simulink model "HouseHeating"  (R2026b)
settings: Solver=FixedStepAuto  StopTime=86400  FixedStep=1  AbsTol=1e-6
InitFcn:
  | sldemo_househeat_data
undefined symbols (not defined in the file): c_air, HeaterAirFlow, LRoof, LWall, LWindow, THeater, TinIC
libraries: fl_lib x22, nesl_utility x4
settings Model: ExtModeTrigMode=oneshot  Creator=The MathWorks, Inc.  LastModifiedBy=jolson
settings SolverCC: AutoScaleAbsTol=off
settings DataIOCC: ExternalInput=[]  InitialState=[]
settings OptimizationCC: BooleansAsBitfields=on  DataBitsets=on  DefaultParameterBehavior=Inlined  DifferentSizesBufferReuse=on  EfficientFloat2IntCast=on  EfficientTunableParamExpr=on  EnhancedBackFolding=on  GainParamInheritBuiltInType=on  InlineInvariantSignals=on  LifeSpan=1  NoFixptDivByZeroProtection=on  OptimizeBlockOrder=speed  PassReuseOutputArgsAs=Individual arguments  RemoveInternalMemoryZeroInit=on  RemoveRootLevelIOMemoryZeroInit=on  StateBitsets=on  UseDivisionForNetSlopeComputation=on  UseFloatMulNetSlope=on
settings DebuggingCC: ArithmeticOperatorsInVariantConditions=warning  BusObjectLabelMismatch=none  FcnCallInpInsideContextMsg=warning  IntegerOverflowMsg=none  IntegerSaturationMsg=none  MergeDetectMultiDrivingBlocksExec=none  MultiTaskCondExecSysMsg=none  MultiTaskDSMMsg=warning  ParameterTunabilityLossMsg=error  SFExecutionAtInitializationDiag=none  SFNoUnconditionalDefaultTransitionDiag=warning  SFUnexpectedBacktrackingDiag=warning  SaveWithParameterizedLinksMsg=none  SignalResolutionControl=TryResolveAllWithWarning  StateNameClashWarn=warning
settings HardwareCC: ProdEndianess=Unspecified  ProdEqTarget=off  ProdHWDeviceType=Generic->32-bit Embedded Processor  ProdIntDivRoundTo=Undefined  ProdLargestAtomicFloat=None  TargetEndianess=LittleEndian  TargetHWDeviceType=MATLAB Host  TargetIntDivRoundTo=Zero  TargetLongLongMode=on
settings ModelReferenceCC: PropagateSignalLabelsOutOfModel=off
settings SFSimCC: CustomCodeUndefinedFunction=UseInterfaceOnly  MATLABDynamicMemAlloc=off  SimUseLocalCustomCode=off
settings RTWCC: DataTypeReplacement=CDataTypesFixedWidth  Description=Embedded Coder  GenerateCodeMetricsReport=on  GenerateReport=on  GenerateTraceInfo=on  GenerateTraceReport=on  GenerateTraceReportEml=on  GenerateTraceReportSf=on  GenerateTraceReportSl=on  IncludeHyperlinkInReport=on  RTWUseLocalCustomCode=off  SystemTargetFile=ert.tlc  TemplateMakefile=ert_default_tmf
settings CodeAppCC: CustomSymbolStrFcn=$N$M$F  CustomSymbolStrGlobalVar=rt$N$M  CustomSymbolStrMacro=$N$M  CustomSymbolStrType=$N$M  ForceParamTrailComments=on  IgnoreCustomStorageClasses=off  InsertBlockDesc=on  OperatorAnnotations=on  SFDataObjDesc=on  SimulinkDataObjDesc=on
settings ERTTargetCC: CombineSignalStateStructs=on  GenerateSampleERTMain=on  MaxIdInt16=INT16_MAX  MaxIdInt32=INT32_MAX  MaxIdInt64=INT64_MAX  MaxIdInt8=INT8_MAX  MaxIdUint16=UINT16_MAX  MaxIdUint32=UINT32_MAX  MaxIdUint64=UINT64_MAX  MaxIdUint8=UINT8_MAX  MinIdInt16=INT16_MIN  MinIdInt32=INT32_MIN  MinIdInt64=INT64_MIN  MinIdInt8=INT8_MIN  SupportContinuousTime=on  SupportNonInlinedSFcns=on  SupportVariableSizeSignals=on
settings ConfigComp: CovExternalEMLEnable=off  CovSaveCumulativeToWorkspaceVar=on  CovSaveSingleToWorkspaceVar=on
settings SimscapeCC: SimscapeNominalValues="[{\"value\":\"1\",\"unit\":\"A\"},{\"value\":\"1\",\"unit\":\"bar\"},{\"value\":\"1\",\"unit\":\"cm^2\"},{\"value\":\"1\",\"unit\":\"cm^3/s\"},{\"value\":\"1\",\"unit\":\"kJ/kg\"},{\"value\":\"1\",\"unit\":\"kW\"},{\"value\":\"1\",\"unit\":\"l\"},{\"value\":\"1\",\"unit\":\"N\"},{\"value\":\"1\",\"unit\":\"N*m\"},{\"value\":\"1\",\"unit\":\"V\"},{\"value\":\"0.001\",\"unit\":\"Wb\"}]"  SimscapeUseEnergyAccounting=off

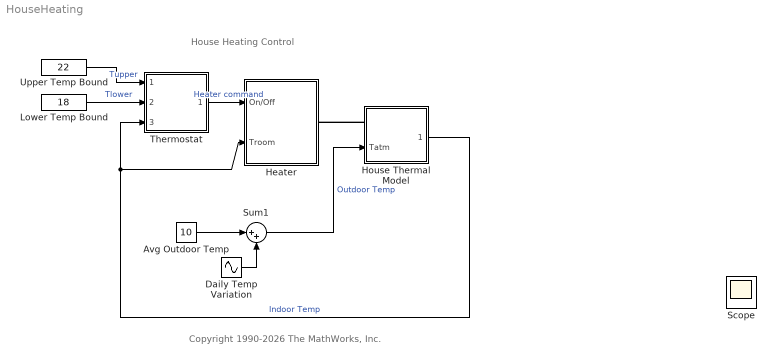
== system HouseHeating ==
  note: House Heating Control
  note: Copyright 1990-2026 The MathWorks, Inc.
  Avg Outdoor Temp : Constant  Value=10
  Daily Temp Variation : Sin  Amplitude=8  Frequency=(2*pi)/(24*3600)  Phase=-pi/2  SampleTime=0
  Heater : Subsystem
  House Thermal Model : Subsystem  Tag=PublishSubsystem
      settings: PortSchema="{\"entries\":[{\"content\":{\"sides\":[{\"content\":{\"connectorIds\":[\"LConn1\",\"In1\"]},\"type\":\"ConnectorPlacement.EquallySpacedRectSide\",\"uuid\":\"eb8069c2-07b2-4f5c-b9f9-5056c4795f4a\"},{\"content\":{\"connectorIds\":[\"Out1\"],\"side\":\"RIGHT\"},\"type\":\"ConnectorPlacement.EquallySpacedRectSide\",\"uuid\":\"80b7e6ec-7098-4e9e-918e-5666993f77ee\"},{\"content\":{\"side\":\"TOP\"},\"type\":\"ConnectorPlacement.EquallySpacedRectSide\",\"uuid\":\"1688e31c-8726-4a54-817f-3a69db3dd392\"}]},\"type\":\"ConnectorPlacement.EquallySpacedConnector\",\"uuid\":\"cc8e1f79-9fa5-412b-9d41-2aa535beff48\"}],\"packageUris\":[\"http://schema.mathworks.com/mf0/Connector/R2020b\"],\"version\":\"1.0\"}"
      mask Display:
      | plot([99.4454661849886;170.309218810871;170.309218810871;99.4454661849886;99.4454661849886], [212.827470386401;212.827470386401;127.790967235342;127.790967235342;212.827470386401])
      | plot([99.4454661849886;170.309218810871], [184.481969336048;184.481969336048])
      | plot([133.460067445412;133.460067445412], [184.481969336048;127.790967235342])
      | plot([241.172971436754;312.036724062636;312.036724062636;241.172971436754;241.172971436754], [212.827470386401;212.827470386401;127.790967235342;127.790967235342;212.827470386401])
      | plot([241.172971436754;312.036724062636], [184.481969336048;184.481969336048])
      | plot([275.187572697178;275.187572697178], [184.481969336048;127.790967235342])
      | plot([113.618216710165;42.7544640842825;368.727726163343;428.253278369084], [453.764229314402;255.34572196193;255.34572196193;453.764229314402])
      | plot([428.253278369084;499.117030994967], [453.764229314402;382.900476688519])
      | plot([113.618216710165;428.253278369084], [453.764229314402;453.764229314402])
      | plot([498.86507098563;499.368991004303], [382.900476688519;382.900476688519])
      | plot([482.109730364755;496.282480889931], [382.900476688519;382.900476688519])
      | plot([482.109730364755;374.396826373413], [382.900476688519;275.187572697178])
      | plot([482.109730364755;425.418728264049], [382.900476688519;439.591478789225])
      | plot([56.927214609459;56.927214609459;354.554975638166], [255.34572196193;56.927214609459;56.927214609459])
      | plot([354.554975638166;354.554975638166], [56.927214609459;255.34572196193])
      | plot([354.554975638166;482.109730364755;482.109730364755], [56.927214609459;184.481969336048;382.900476688519])
      | plot([397.073227213696;397.073227213696;439.591478789225;439.591478789225;397.073227213696], [170.309218810871;255.34572196193;297.86397353746;209.992920281366;170.309218810871])
      | plot([397.073227213696;439.591478789225], [227.000220911577;269.518472487107])
      | plot([419.749628053978;419.749628053978], [246.842071646824;192.985619651154])
      | %patch([0;553.20969549939;553.20969549939;0;0;0.472425017505884;0.47242501750577;552.737270481884;552.737270481885;0.472425017505884;0], [496.518693398684;496.518693398684;0;0;496.518693398684;496.046268381178;0.472425017505884;0.472425017505884;496.046268381178;496.046268381178;496.518693398684], [1;1;1])
  Lower Temp Bound : Constant  Value=18
  Sum1 : Sum  Inputs=|++  InputSameDT=on  SaturateOnIntegerOverflow=on  OutDataTypeStr=Inherit: Same as first input
  Thermostat : Subsystem
  Upper Temp Bound : Constant  Value=22
  Scope : Scope
      settings: ActiveDisplayYMinimum=-0.49999999999999956  ActiveDisplayYMaximum=24.5
  wires:
  Thermostat/1(HeaterSwitch) -> Heater/1(On/Off)  "Heater command"
  Daily Temp Variation/1 -> Sum1/2
  Sum1/1 -> House Thermal Model/1(Tatm)  "Outdoor Temp"
  Avg Outdoor Temp/1 -> Sum1/1
  House Thermal Model/1(Troom) -> Thermostat/3(Thouse), Heater/2(Troom)  "Indoor Temp"
  Lower Temp Bound/1 -> Thermostat/2(Tlower)  "Tlower"
  Upper Temp Bound/1 -> Thermostat/1(Tupper)  "Tupper"
  connections:
  House Thermal Model/LConn1 -- Heater/RConn1

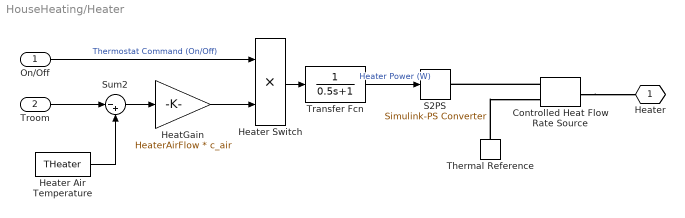
== system HouseHeating/Heater ==
  On/Off : Inport
  Troom : Inport  Port=2
  Controlled Heat Flow Rate Source : fl_lib/Thermal/Thermal Sources/Controlled Heat Flow Rate Source
  HeatGain : Gain  Gain=HeaterAirFlow * c_air
  Heater Air Temperature : Constant  Value=THeater
  Heater Switch : Product  RndMeth=Zero
  S2PS : nesl_utility/Simulink-PS Converter  PhysicalDomain=network_engine_domain  SubClassName=ps_input  LeftPortType=input  RightPortType=output  PseudoPeriodic=off  Frequencies=[]  NoiseDistribution=none  NoiseParameters=[]  Unit=1  AffineConversion=off  FilteringAndDerivatives=zero  SimscapeFilterOrder=1  InputFilterTimeConstant=.001  UdotUserProvided=0
  Sum2 : Sum  Inputs=|-+
  Thermal Reference : fl_lib/Thermal/Thermal Elements/Thermal Reference
  Transfer Fcn : TransferFcn  Denominator=[0.5 1]
  Heater : PMIOPort  Tag=PMCPort  Side=Right
  wires:
  Heater Air Temperature/1 -> Sum2/2
  Troom/1 -> Sum2/1
  Sum2/1 -> HeatGain/1
  On/Off/1 -> Heater Switch/1  "Thermostat Command (On/Off)"
  HeatGain/1 -> Heater Switch/2
  Heater Switch/1 -> Transfer Fcn/1
  Transfer Fcn/1 -> S2PS/1  "Heater Power (W)"
  connections:
  Controlled Heat Flow Rate Source/RConn1 -- S2PS/RConn1
  Thermal Reference/LConn1 -- Controlled Heat Flow Rate Source/RConn2
  Controlled Heat Flow Rate Source/LConn1 -- Heater/RConn1

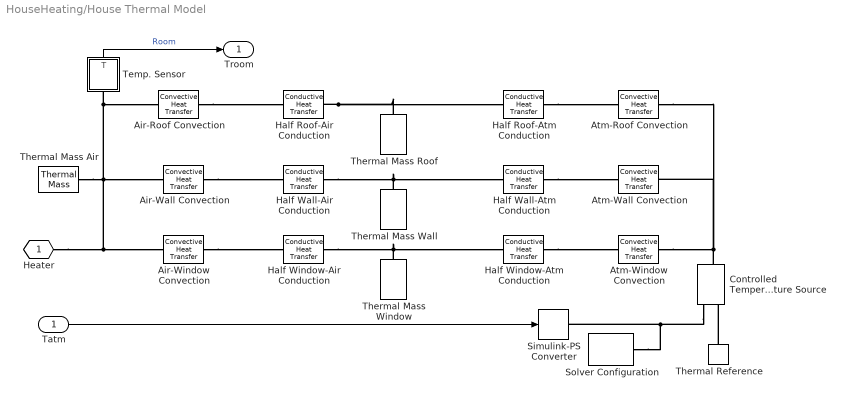
== system HouseHeating/House Thermal Model ==
  Tatm : Inport
  Air-Roof Convection : fl_lib/Thermal/Thermal Elements/Convective Heat Transfer  thermal_type=foundation.enum.constant_variable.constant  area=roofArea m^2  heat_tr_coeff=h_A_R W/m^2/K  min_heat_tr_coeff=1e-3 W/(K*m^2)  T_specify=off  T_priority=High  T=0 K  T_nominal_specify=off  T_nominal_value=1  T_nominal_unit=K  Q_specify=off  Q_priority=High  Q=0 J/s  Q_nominal_specify=off  Q_nominal_value=1  Q_nominal_unit=W
  Air-Wall Convection : fl_lib/Thermal/Thermal Elements/Convective Heat Transfer  thermal_type=foundation.enum.constant_variable.constant  area=wallArea m^2  heat_tr_coeff=h_A_W W/m^2/K  min_heat_tr_coeff=1e-3 W/(K*m^2)  T_specify=off  T_priority=High  T=0 K  T_nominal_specify=off  T_nominal_value=1  T_nominal_unit=K  Q_specify=off  Q_priority=High  Q=0 J/s  Q_nominal_specify=off  Q_nominal_value=1  Q_nominal_unit=W
  Air-Window Convection : fl_lib/Thermal/Thermal Elements/Convective Heat Transfer  thermal_type=foundation.enum.constant_variable.constant  area=windowArea m^2  heat_tr_coeff=h_A_Wnd W/m^2/K  min_heat_tr_coeff=1e-3 W/(K*m^2)  T_specify=off  T_priority=High  T=0 K  T_nominal_specify=off  T_nominal_value=1  T_nominal_unit=K  Q_specify=off  Q_priority=High  Q=0 J/s  Q_nominal_specify=off  Q_nominal_value=1  Q_nominal_unit=W
  Atm-Roof Convection : fl_lib/Thermal/Thermal Elements/Convective Heat Transfer  thermal_type=foundation.enum.constant_variable.constant  area=roofArea m^2  heat_tr_coeff=h_R_Atm W/m^2/K  min_heat_tr_coeff=1e-3 W/(K*m^2)  T_specify=off  T_priority=High  T=0 K  T_nominal_specify=off  T_nominal_value=1  T_nominal_unit=K  Q_specify=off  Q_priority=High  Q=0 J/s  Q_nominal_specify=off  Q_nominal_value=1  Q_nominal_unit=W
  Atm-Wall Convection : fl_lib/Thermal/Thermal Elements/Convective Heat Transfer  thermal_type=foundation.enum.constant_variable.constant  area=wallArea m^2  heat_tr_coeff=h_W_Atm W/m^2/K  min_heat_tr_coeff=1e-3 W/(K*m^2)  T_specify=off  T_priority=High  T=0 K  T_nominal_specify=off  T_nominal_value=1  T_nominal_unit=K  Q_specify=off  Q_priority=High  Q=0 J/s  Q_nominal_specify=off  Q_nominal_value=1  Q_nominal_unit=W
  Atm-Window Convection : fl_lib/Thermal/Thermal Elements/Convective Heat Transfer  thermal_type=foundation.enum.constant_variable.constant  area=windowArea m^2  heat_tr_coeff=h_Wnd_Atm W/m^2/K  min_heat_tr_coeff=1e-3 W/(K*m^2)  T_specify=off  T_priority=High  T=0 K  T_nominal_specify=off  T_nominal_value=1  T_nominal_unit=K  Q_specify=off  Q_priority=High  Q=0 J/s  Q_nominal_specify=off  Q_nominal_value=1  Q_nominal_unit=W
  Controlled Temperature Source : fl_lib/Thermal/Thermal Sources/Controlled Temperature Source
  Half Roof-Air Conduction : fl_lib/Thermal/Thermal Elements/Conductive Heat Transfer  thermal_type=foundation.enum.ConstantVariableTabulated.Constant  wall_geometry=foundation.enum.ConductionWallGeometry.Planar  area=roofArea m^2  thickness=LRoof/2 m  d_in=0.05 m  d_out=0.1 m  L=1 m  th_cond_min=10 W/(K*m)  th_cond=kRoof W/m/K  th_cond_TLU=[413, 401, 392, 383, 371, 357, 342] W/(K*m)  temp_TLU=[200, 273, 400, 600, 800, 1000, 1200] K  T_specify=off  T_priority=High  T=0 K  T_nominal_specify=off  T_nominal_value=1  T_nominal_unit=K  Q_specify=off  Q_priority=High  Q=0 J/s  Q_nominal_specify=off  Q_nominal_value=1  Q_nominal_unit=W
  Half Roof-Atm Conduction : fl_lib/Thermal/Thermal Elements/Conductive Heat Transfer  thermal_type=foundation.enum.ConstantVariableTabulated.Constant  wall_geometry=foundation.enum.ConductionWallGeometry.Planar  area=roofArea m^2  thickness=LRoof/2 m  d_in=0.05 m  d_out=0.1 m  L=1 m  th_cond_min=10 W/(K*m)  th_cond=kRoof W/m/K  th_cond_TLU=[413, 401, 392, 383, 371, 357, 342] W/(K*m)  temp_TLU=[200, 273, 400, 600, 800, 1000, 1200] K  T_specify=off  T_priority=High  T=0 K  T_nominal_specify=off  T_nominal_value=1  T_nominal_unit=K  Q_specify=off  Q_priority=High  Q=0 J/s  Q_nominal_specify=off  Q_nominal_value=1  Q_nominal_unit=W
  Half Wall-Air Conduction : fl_lib/Thermal/Thermal Elements/Conductive Heat Transfer  thermal_type=foundation.enum.ConstantVariableTabulated.Constant  wall_geometry=foundation.enum.ConductionWallGeometry.Planar  area=wallArea m^2  thickness=LWall/2 m  d_in=0.05 m  d_out=0.1 m  L=1 m  th_cond_min=10 W/(K*m)  th_cond=kWall W/m/K  th_cond_TLU=[413, 401, 392, 383, 371, 357, 342] W/(K*m)  temp_TLU=[200, 273, 400, 600, 800, 1000, 1200] K  T_specify=off  T_priority=High  T=0 K  T_nominal_specify=off  T_nominal_value=1  T_nominal_unit=K  Q_specify=off  Q_priority=High  Q=0 J/s  Q_nominal_specify=off  Q_nominal_value=1  Q_nominal_unit=W
  Half Wall-Atm Conduction : fl_lib/Thermal/Thermal Elements/Conductive Heat Transfer  thermal_type=foundation.enum.ConstantVariableTabulated.Constant  wall_geometry=foundation.enum.ConductionWallGeometry.Planar  area=wallArea m^2  thickness=LWall/2 m  d_in=0.05 m  d_out=0.1 m  L=1 m  th_cond_min=10 W/(K*m)  th_cond=kWall W/m/K  th_cond_TLU=[413, 401, 392, 383, 371, 357, 342] W/(K*m)  temp_TLU=[200, 273, 400, 600, 800, 1000, 1200] K  T_specify=off  T_priority=High  T=0 K  T_nominal_specify=off  T_nominal_value=1  T_nominal_unit=K  Q_specify=off  Q_priority=High  Q=0 J/s  Q_nominal_specify=off  Q_nominal_value=1  Q_nominal_unit=W
  Half Window-Air Conduction : fl_lib/Thermal/Thermal Elements/Conductive Heat Transfer  thermal_type=foundation.enum.ConstantVariableTabulated.Constant  wall_geometry=foundation.enum.ConductionWallGeometry.Planar  area=windowArea m^2  thickness=LWindow/2 m  d_in=0.05 m  d_out=0.1 m  L=1 m  th_cond_min=10 W/(K*m)  th_cond=kWindow W/m/K  th_cond_TLU=[413, 401, 392, 383, 371, 357, 342] W/(K*m)  temp_TLU=[200, 273, 400, 600, 800, 1000, 1200] K  T_specify=off  T_priority=High  T=0 K  T_nominal_specify=off  T_nominal_value=1  T_nominal_unit=K  Q_specify=off  Q_priority=High  Q=0 J/s  Q_nominal_specify=off  Q_nominal_value=1  Q_nominal_unit=W
  Half Window-Atm Conduction : fl_lib/Thermal/Thermal Elements/Conductive Heat Transfer  thermal_type=foundation.enum.ConstantVariableTabulated.Constant  wall_geometry=foundation.enum.ConductionWallGeometry.Planar  area=windowArea m^2  thickness=LWindow/2 m  d_in=0.05 m  d_out=0.1 m  L=1 m  th_cond_min=10 W/(K*m)  th_cond=kWindow W/m/K  th_cond_TLU=[413, 401, 392, 383, 371, 357, 342] W/(K*m)  temp_TLU=[200, 273, 400, 600, 800, 1000, 1200] K  T_specify=off  T_priority=High  T=0 K  T_nominal_specify=off  T_nominal_value=1  T_nominal_unit=K  Q_specify=off  Q_priority=High  Q=0 J/s  Q_nominal_specify=off  Q_nominal_value=1  Q_nominal_unit=W
  Simulink-PS Converter : nesl_utility/Simulink-PS Converter  PhysicalDomain=network_engine_domain  SubClassName=ps_input  LeftPortType=input  RightPortType=output  PseudoPeriodic=off  Frequencies=[]  NoiseDistribution=none  NoiseParameters=[]  Unit=degC  AffineConversion=on  FilteringAndDerivatives=zero  SimscapeFilterOrder=1  InputFilterTimeConstant=.001  UdotUserProvided=0
  Solver Configuration : nesl_utility/Solver Configuration  PhysicalDomain=network_engine_domain  SubClassName=solver  LeftPortType=input  RightPortType=generic  Tones=[]  Harmonics=[]  SimulateNoise=off  Profile=off  UseLocalSampling=off  EnableSwitchedLinearOptims=on  FrequencyDomain=off  UseCCode=off  RelTol=0.001  AbsTol=1e-06  MinStep=1e-09  ToWorkspace=off  RevertToSquareIcSolve=off  NumHomotopyIterations=100  PhasorMode=off  PhasorModeNumHarmonics=1  ConsistencySolver=NEWTON_XTOL_AFTER_FTOL  CanonicalOrdering=UNORDERED  OptimizeIntermediates=UNOPTIMIZED  MulticoreSolverChoice=BACKWARD_EULER  IndexReductionMethod=DerivativeReplacement  DoDC=off  ResidualTolerance=1e-9  ConsistencyTolSource=GLOBAL  ConsistencyAbsTol=0.001  ConsistencyRelTol=0.001  ConsistencyTolFactor=0.001  UseLocalSolver=off  LocalSolverChoice=NE_BACKWARD_EULER_ADVANCER  ResolveIndetEquations=on  FunctionEvalNumThread=1  LocalSolverSampleTime=.001  DoFixedCost=off  MaxNonlinIter=3  MaxModeIter=2  ComputeImpulses=off  ImpulseIterations=2  LinearAlgebra=auto  LinearAlgebraNumThread=0  EquationFormulation=NE_TIME_EF  DelaysMemoryBudget=1024  AutomaticFiltering=on  FilteringTimeConstant=0.001  PartitionStorageMethod=AS_NEEDED  PartitionMemoryBudget=1024  PartitionMethod=FAST  MultibodyUseLocalSolver=off  MultibodyLocalSolverChoice=ODE1  MultibodyLocalSolverSampleTime=0.001
  Temp. Sensor : Subsystem
  Thermal Mass Air : fl_lib/Thermal/Thermal Elements/Thermal Mass  mass_type=foundation.enum.constant_variable.constant  mass=M_air kg  sp_heat=c_air J/kg/K  mass_min=1e-6 kg  num_ports=foundation.enum.numPorts2.one  m_specify=off  m_priority=High  m=1 kg  m_nominal_specify=off  m_nominal_value=1  m_nominal_unit=kg  T_specify=on  T_priority=High  T=TinIC degC  T_nominal_specify=off  T_nominal_value=1  T_nominal_unit=K  Q_specify=off  Q_priority=None  Q=0 W  Q_nominal_specify=off  Q_nominal_value=1  Q_nominal_unit=W
  Thermal Mass Roof : fl_lib/Thermal/Thermal Elements/Thermal Mass  mass_type=foundation.enum.constant_variable.constant  mass=roofMass kg  sp_heat=c_roof J/kg/K  mass_min=1e-6 kg  num_ports=foundation.enum.numPorts2.one  m_specify=off  m_priority=High  m=1 kg  m_nominal_specify=off  m_nominal_value=1  m_nominal_unit=kg  T_specify=on  T_priority=High  T=TinIC degC  T_nominal_specify=off  T_nominal_value=1  T_nominal_unit=K  Q_specify=off  Q_priority=None  Q=0 W  Q_nominal_specify=off  Q_nominal_value=1  Q_nominal_unit=W
  Thermal Mass Wall : fl_lib/Thermal/Thermal Elements/Thermal Mass  mass_type=foundation.enum.constant_variable.constant  mass=wallMass kg  sp_heat=c_wall J/kg/K  mass_min=1e-6 kg  num_ports=foundation.enum.numPorts2.one  m_specify=off  m_priority=High  m=1 kg  m_nominal_specify=off  m_nominal_value=1  m_nominal_unit=kg  T_specify=on  T_priority=High  T=TinIC degC  T_nominal_specify=off  T_nominal_value=1  T_nominal_unit=K  Q_specify=off  Q_priority=None  Q=0 W  Q_nominal_specify=off  Q_nominal_value=1  Q_nominal_unit=W
  Thermal Mass Window : fl_lib/Thermal/Thermal Elements/Thermal Mass  mass_type=foundation.enum.constant_variable.constant  mass=windowMass kg  sp_heat=c_window J/kg/K  mass_min=1e-6 kg  num_ports=foundation.enum.numPorts2.one  m_specify=off  m_priority=High  m=1 kg  m_nominal_specify=off  m_nominal_value=1  m_nominal_unit=kg  T_specify=on  T_priority=High  T=TinIC degC  T_nominal_specify=off  T_nominal_value=1  T_nominal_unit=K  Q_specify=off  Q_priority=None  Q=0 W  Q_nominal_specify=off  Q_nominal_value=1  Q_nominal_unit=W
  Thermal Reference : fl_lib/Thermal/Thermal Elements/Thermal Reference
  Heater : PMIOPort  Tag=PMCPort  Side=Left
  Troom : Outport  VectorParamsAs1DForOutWhenUnconnected=off
  wires:
  Tatm/1 -> Simulink-PS Converter/1
  Temp. Sensor/1(T) -> Troom/1  "Room"
  connections:
  Thermal Reference/LConn1 -- Controlled Temperature Source/RConn2
  Solver Configuration/RConn1 -- Controlled Temperature Source/RConn1 -- Simulink-PS Converter/RConn1
  Heater/RConn1 -- Air-Window Convection/LConn1 -- Thermal Mass Air/LConn1 -- Air-Wall Convection/LConn1 -- Air-Roof Convection/LConn1 -- Temp. Sensor/LConn1
  Air-Wall Convection/RConn1 -- Half Wall-Air Conduction/LConn1
  Half Wall-Air Conduction/RConn1 -- Thermal Mass Wall/LConn1 -- Half Wall-Atm Conduction/LConn1
  Half Wall-Atm Conduction/RConn1 -- Atm-Wall Convection/LConn1
  Air-Window Convection/RConn1 -- Half Window-Air Conduction/LConn1
  Half Window-Air Conduction/RConn1 -- Thermal Mass Window/LConn1 -- Half Window-Atm Conduction/LConn1
  Half Window-Atm Conduction/RConn1 -- Atm-Window Convection/LConn1
  Air-Roof Convection/RConn1 -- Half Roof-Air Conduction/LConn1
  Half Roof-Air Conduction/RConn1 -- Half Roof-Atm Conduction/LConn1 -- Thermal Mass Roof/LConn1
  Half Roof-Atm Conduction/RConn1 -- Atm-Roof Convection/LConn1
  Atm-Window Convection/RConn1 -- Controlled Temperature Source/LConn1 -- Atm-Roof Convection/RConn1 -- Atm-Wall Convection/RConn1

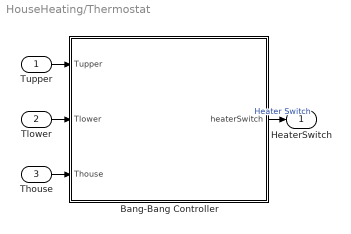
== system HouseHeating/Thermostat ==
  Tupper : Inport
  Tlower : Inport  Port=2
  Thouse : Inport  Port=3
  Bang-Bang Controller : Stateflow chart  TreatAsAtomicUnit=on  SystemSampleTime=300
      settings: PortSchema="{\"entries\":[{\"content\":{\"sides\":[{\"content\":{\"connectorIds\":[\"In2\",\"In1\",\"In3\"]},\"type\":\"ConnectorPlacement.EquallySpacedRectSide\",\"uuid\":\"e68fab5f-d8fa-402f-98f2-b30b767afde8\"},{\"content\":{\"connectorIds\":[\"Out1\"],\"side\":\"RIGHT\"},\"type\":\"ConnectorPlacement.EquallySpacedRectSide\",\"uuid\":\"6bda6de8-a23e-4749-a421-1fa501b9d401\"},{\"content\":{\"side\":\"TOP\"},\"type\":\"ConnectorPlacement.EquallySpacedRectSide\",\"uuid\":\"87edbce4-be3e-425d-8538-3e8fde7c19d0\"}]},\"type\":\"ConnectorPlacement.EquallySpacedConnector\",\"uuid\":\"d94f3911-5cd5-49ee-9855-90a29033781c\"}],\"packageUris\":[\"http://schema.mathworks.com/mf0/Connector/R2020b\"],\"version\":\"1.0\"}"
  HeaterSwitch : Outport  InitialOutput=0  VectorParamsAs1DForOutWhenUnconnected=off
  wires:
  Bang-Bang Controller/1(heaterSwitch) -> HeaterSwitch/1  "Heater Switch"
  Tlower/1 -> Bang-Bang Controller/1(Tlower)
  Thouse/1 -> Bang-Bang Controller/3(Thouse)
  Tupper/1 -> Bang-Bang Controller/2(Tupper)

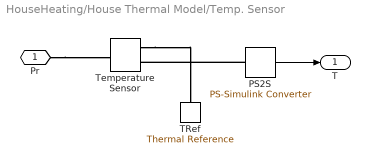
== system HouseHeating/House Thermal Model/Temp. Sensor ==
  PS2S : nesl_utility/PS-Simulink Converter  PhysicalDomain=network_engine_domain  SubClassName=ps_output  LeftPortType=input  RightPortType=output  PseudoPeriodic=off  Frequencies=[]  VectorFormat=1-D array  Unit=degC  AffineConversion=on
  TRef : fl_lib/Thermal/Thermal Elements/Thermal Reference
  Temperature Sensor : fl_lib/Thermal/Thermal Sensors/Temperature Sensor  temperature_measure=foundation.enum.MeasurementReference.difference
  Pr : PMIOPort  Side=Left
  T : Outport  VectorParamsAs1DForOutWhenUnconnected=off
  wires:
  PS2S/1 -> T/1
  connections:
  Temperature Sensor/RConn1 -- TRef/LConn1
  PS2S/LConn1 -- Temperature Sensor/RConn2
  Pr/RConn1 -- Temperature Sensor/LConn1

== stateflow chart HouseHeating/Thermostat/Bang-Bang Controller ==
  state Heater_On
    during:
    heaterSwitch = true;
  state Heater_Off
    during:
    heaterSwitch = false;
  (default) -> Heater_Off
  Heater_On -> Heater_Off : % Switch with 0.2 degree headroom
      | [Thouse>=(Tupper-0.2)]
  Heater_Off -> Heater_On : % Switch with 0.2 degree headroom
      | [Thouse<=Tlower]
  data: heaterSwitch output; Tlower input =2; Tupper input; Thouse input
